simulink model "IM_DRIVE"  (R2025a)
settings: Solver=FixedStepDiscrete  StartTime=0.0  StopTime=scen.Tend  FixedStep=P.ctrl.Ts  RelTol=1e-3
undefined symbols (not defined in the file or in its folder): P
settings Model: Creator=ironman  LastModifiedBy=ironman
settings DataIOCC: SaveOutput=off  SignalLogging=off  SaveTime=off

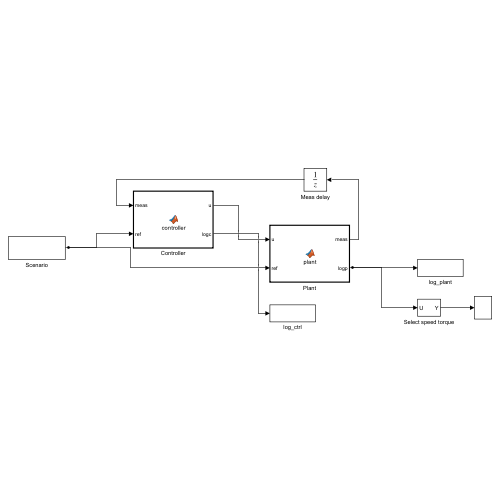
[thumbnail: Simulink's stored preview of the top-level diagram]
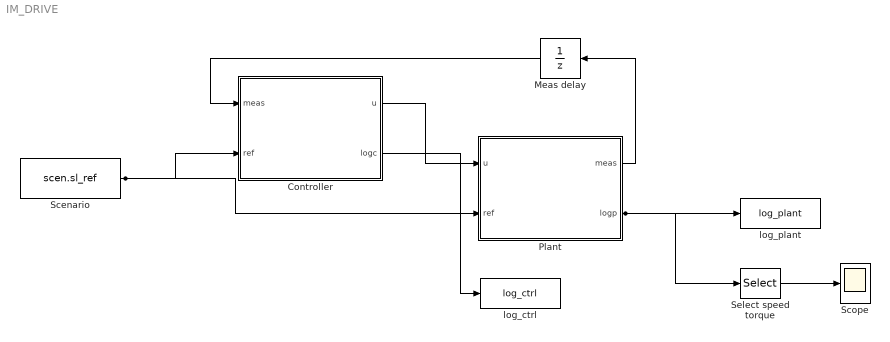
== system IM_DRIVE ==
  Controller : MATLAB Function  TreatAsAtomicUnit=on
  Meas delay : UnitDelay  InitialCondition=zeros(4,1)  SampleTime=P.ctrl.Ts  HasFrameUpgradeWarning=on
  Plant : MATLAB Function  TreatAsAtomicUnit=on
  Scenario : FromWorkspace  VariableName=scen.sl_ref  SampleTime=P.ctrl.Ts  Interpolate=off  OutputAfterFinalValue=Holding final value
  Scope : Scope
  Select speed torque : Selector  InputPortWidth=23  IndexOptions=Index vector (dialog)  Indices=[4 5]  OutputSizes=1
  log_ctrl : ToWorkspace  VariableName=log_ctrl  SaveFormat=Structure With Time  SampleTime=-1
      settings: Decimation=P.sim.log_decim
  log_plant : ToWorkspace  VariableName=log_plant  SaveFormat=Structure With Time  SampleTime=-1
      settings: Decimation=P.sim.log_decim
  wires:
  Scenario/1 -> Controller/2(ref), Plant/2(ref)
  Controller/1(u) -> Plant/1(u)
  Plant/1(meas) -> Meas delay/1
  Meas delay/1 -> Controller/1(meas)
  Plant/2(logp) -> log_plant/1, Select speed torque/1
  Controller/2(logc) -> log_ctrl/1
  Select speed torque/1 -> Scope/1

== matlab function IM_DRIVE/Plant ==
  data: u input; meas output; ref input; logp output; P parameter
function [meas, logp] = plant(u, ref, P)
%#codegen
% Two-level inverter + saturated induction motor (see core/plant_step.m)
persistent pst
if isempty(pst)
    pst = plant_init(P);
end
[meas, logp, pst] = plant_step(pst, u, ref, P);

== matlab function IM_DRIVE/Controller ==
  data: meas input; u output; ref input; logc output; P parameter
function [u, logc] = controller(meas, ref, P)
%#codegen
% Drive controller: IFOC or DTC selected by P.ctrl.type (see core/ctrl_step.m)
persistent st
if isempty(st)
    st = ctrl_init(P);
end
[u, logc, st] = ctrl_step(st, meas, ref, P);
